simulink model "LMCL"  (R2024b)
settings: Solver=ode4  StartTime=0  StopTime=300  FixedStep=0.01  RelTol=1e-3  AbsTol=1e-6
values from neighbouring files (symbols this model uses):
  C_Alt = pidtune(G_Fz2Alt,'pdf',1)    [controller.m]
  C_phi = pidtune(G_Mx2phi,'pdf',wc)    [controller.m]
  C_psi = pidtune(G_Mz2psi,'pdf',wc)    [controller.m]
  C_tht = pidtune(G_My2tht,'pdf',wc)    [controller.m]
  C_Vx = pidtune(-G_Fx2Vx,'p',0.05)    [controller.m]
  C_Vy = pidtune(-G_Fy2Vy,'p',0.08)    [controller.m]
  C_Vz = pidtune(G_Fz2Vz,'pi',0.05)    [controller.m]
  Ixx = 135582    [initialization.m]
  Iyy = 149140.0    (= 149140)    [initialization.m]
  Izz = 135582    [initialization.m]
  lat_grid = linspace(-90, 90, num_lat)    [initialization.m]
  lon_grid = linspace(-180, 180, num_lon)    [initialization.m]
  moon_dem_table = flipud(raw_data)    [initialization.m]
undefined symbols (not defined in the file or in its folder): datetime, gray, juliandate, Sim3dSensor
libraries: slpidlib x7, sim3dcameralib x3, sim3dlib x2, simulink x2, aerolibtransform2 x2, sharedtransform x1
Description:
  | Apollo Lunar Module Digital Autopilot
settings Model: RequirementInfo=9  SimulationMode=accelerator  PacingRate=1000  Creator=The MathWorks, Inc.  LastModifiedBy=abdma
settings SolverCC: AutoScaleAbsTol=off  AlgebraicLoopSolver=TrustRegion  MaxZcPerStep=1
settings DataIOCC: ExternalInput=op  InitialState=op  SaveFormat=Array  ReturnWorkspaceOutputs=off  SignalLoggingName=logsOut
settings OptimizationCC: BlockReduction=off  ExpressionDepthLimit=2147483647  InitFltsAndDblsToZero=on
settings DebuggingCC: SaveWithParameterizedLinksMsg=none  SignalResolutionControl=TryResolveAllWithWarning  MultiTaskDSMMsg=warning  MultiTaskCondExecSysMsg=none  SigSpecEnsureSampleTimeMsg=none  FcnCallInpInsideContextMsg=warning  UnconnectedInputMsg=warning  UnconnectedOutputMsg=warning  UnconnectedLineMsg=warning  StateNameClashWarn=warning  SFUnexpectedBacktrackingDiag=warning  SFNoUnconditionalDefaultTransitionDiag=warning  SFExecutionAtInitializationDiag=none  ArithmeticOperatorsInVariantConditions=warning
settings HardwareCC: ProdBitPerPointer=32  ProdBitPerSizeT=32  ProdBitPerPtrDiffT=32  ProdLargestAtomicFloat=None  ProdIntDivRoundTo=Undefined  ProdEndianess=Unspecified  ProdWordSize=32  ProdHWDeviceType=Specified
settings ModelReferenceCC: EnableRefExpFcnMdlSchedulingChecks=on  PropagateSignalLabelsOutOfModel=off
settings SFSimCC: SimUseLocalCustomCode=off  SimParseCustomCode=off  CustomCodeUndefinedFunction=UseInterfaceOnly
settings RTWCC: RTWUseLocalCustomCode=off  GPUComputeCapability=3.5  DLArmComputeVersion=19.05
settings CodeAppCC: StateflowObjectComments=on
settings GRTTargetCC: TargetLangStandard=C89/C90 (ANSI)
settings ConfigComp: CovMetricSettings=d  CovSaveCumulativeToWorkspaceVar=on  CovSaveSingleToWorkspaceVar=on  CovExternalEMLEnable=off

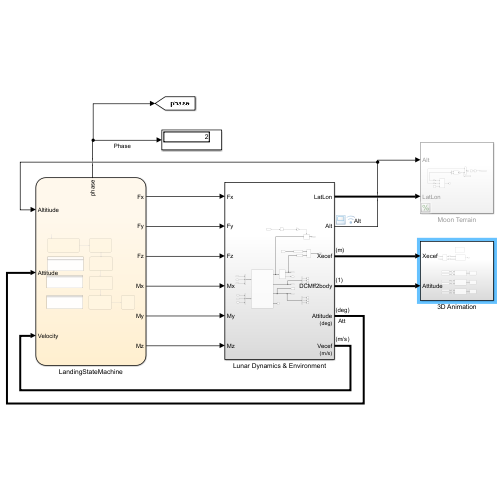
[thumbnail: Simulink's stored preview of the top-level diagram]
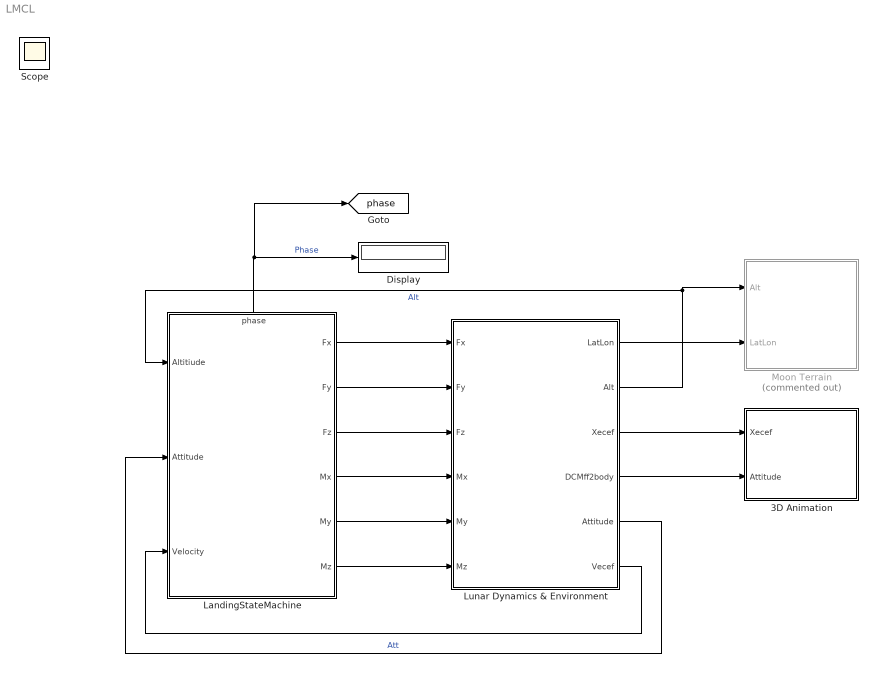
== system LMCL ==
  3D Animation : Subsystem
  Display : Display
  LandingStateMachine : Stateflow chart  TreatAsAtomicUnit=on
      settings: PortSchema="{\"entries\":[{\"content\":{\"sides\":[{\"content\":{\"connectorIds\":[\"In2\",\"In1\",\"In3\"]},\"type\":\"ConnectorPlacement.EquallySpacedRectSide\",\"uuid\":\"b70f077f-5e53-4c11-8b70-291da90a2e92\"},{\"content\":{\"connectorIds\":[\"Out1\",\"Out2\",\"Out3\",\"Out4\",\"Out5\",\"Out6\"],\"side\":\"RIGHT\"},\"type\":\"ConnectorPlacement.EquallySpacedRectSide\",\"uuid\":\"64878038-02c9-47ce-a3b0-eea076ce4bef\"},{\"content\":{\"connectorIds\":[\"Out7\"],\"side\":\"TOP\"},\"type\":\"ConnectorPlacement.EquallySpacedRectSide\",\"uuid\":\"8f914426-e7c7-4385-9703-b406b77ddbb5\"},{\"content\":{\"side\":\"BOTTOM\"},\"type\":\"ConnectorPlacement.EquallySpacedRectSide\",\"uuid\":\"32269b0d-665b-4735-ae33-dac0ab7999d4\"}]},\"type\":\"ConnectorPlacement.EquallySpacedConnector\",\"uuid\":\"201aca57-d29b-4529-a69e-c761b29ced2a\"}],\"packageUris\":[\"http://schema.mathworks.com/mf0/Connector/R2020b\"],\"version\":\"1.0\"}"
  Lunar Dynamics & Environment : Subsystem
  Moon Terrain : Subsystem  Commented=on
  Scope : Scope
  tag scope: phase=global
  wires:
  Lunar Dynamics & Environment/2(Alt) -> LandingStateMachine/2(Altitiude), Moon Terrain/1(Alt)  "Alt"
  Lunar Dynamics & Environment/6(Vecef) -> LandingStateMachine/3(Velocity)
  Lunar Dynamics & Environment/5(Attitude) -> LandingStateMachine/1(Attitude)  "Att"
  LandingStateMachine/1(Fx) -> Lunar Dynamics & Environment/1(Fx)
  LandingStateMachine/2(Fy) -> Lunar Dynamics & Environment/2(Fy)
  LandingStateMachine/3(Fz) -> Lunar Dynamics & Environment/3(Fz)
  LandingStateMachine/4(Mx) -> Lunar Dynamics & Environment/4(Mx)
  LandingStateMachine/5(My) -> Lunar Dynamics & Environment/5(My)
  LandingStateMachine/6(Mz) -> Lunar Dynamics & Environment/6(Mz)
  LandingStateMachine/7(phase) -> [phase], Display/1  "Phase"
  Lunar Dynamics & Environment/1(LatLon) -> Moon Terrain/2(LatLon)
  Lunar Dynamics & Environment/3(Xecef) -> 3D Animation/1(Xecef)
  Lunar Dynamics & Environment/4(DCMff2body) -> 3D Animation/2(Attitude)

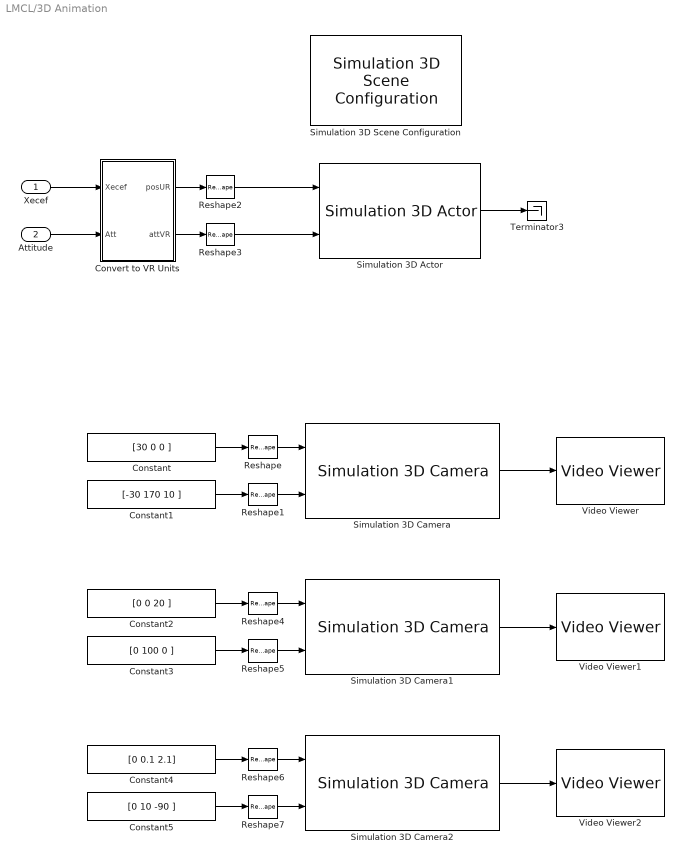
== system LMCL/3D Animation ==
  Xecef : Inport
  Attitude : Inport  Port=2
  Constant : Constant  Value=[30 0 0 ]
  Constant1 : Constant  Value=[-30 170 10 ]
  Constant2 : Constant  Value=[0 0 20 ]
  Constant3 : Constant  Value=[0 100 0 ]
  Constant4 : Constant  Value=[0 0.1 2.1]
  Constant5 : Constant  Value=[0 10 -90 ]
  Convert to VR Units : Subsystem
  Reshape{,1..7} (8 alike) : Reshape  OutputDimensionality=Customize  OutputDimensions=[1,3]
  Simulation 3D Actor : sim3dlib/Simulation 3D Actor  Priority=1  ActorName=LunarModule  ParentName=Scene Origin  Operation=Create at setup  InitScriptText=|  SampleTime=-1  Translation=[10000 10000 10000]  Rotation=[0 0 0]  Scale=[1 1 1]  InputsText=LunarModule.Translation LunarModule.Rotation  aMode=5  ActorTag=LunarModule  ActorType=Sim3dActor  ID=C
      | % Initialize actor
      | Actor.Physics = true;
      | 
      | % Camera that outputs images (optional)
      | camera1 = sim3d.sensors.IdealCamera( ...
      |     'ActorName',"Camera1", ...
      |     "ImageSize",[768, 1024], ...
      |     "HorizontalFieldOfView",60);
      | camera1.Translation = [-3 0 2];
      | add(World, camera1);
      | 
      | % Viewport: this is what changes the view you see
      | createViewport(World, Translation=[-5 0 1], Rotation=[0 0 0]);
  Simulation 3D Camera : sim3dcameralib/Simulation 3D Camera  Priority=1  sensorTag=Sim3dSensor�  sensorId=1  sensorName=Sim3dSensor�  vehTagList={'LunarModule';'Scene Origin'}  vehTag=LunarModule  mountLoc=Origin  offsetFlag=on  tmountOffset=[0, 0, 0]  extTmount=on  rmountOffset=[0, 0, 0]  extRmount=on  FocalLength=[1109, 1109]  OpticalCenter=[640, 360]  ImageSize=[720, 1280]  RadialDistortion=[0, 0]  TangentialDistortion=[0, 0]  SensorSkew=0  DepthOutportEnabled=off  SemanticOutportEnabled=off  TransformOutportEnabled=off  SampleTime=-1  mountPoint=[0 0 0]  mountOrientation=[0 0 0]  aMode=3  ID=1
      settings: LibrarySourceBlock=drivingsim3d/Simulation 3D Camera
  Simulation 3D Camera1 : sim3dcameralib/Simulation 3D Camera  Priority=1  sensorTag=Sim3dSensor�  sensorId=2  sensorName=Sim3dSensor�  vehTagList={'LunarModule';'Scene Origin'}  vehTag=LunarModule  mountLoc=Origin  offsetFlag=on  tmountOffset=[0, 0, 0]  extTmount=on  rmountOffset=[0, 0, 0]  extRmount=on  FocalLength=[1109, 1109]  OpticalCenter=[640, 360]  ImageSize=[720, 1280]  RadialDistortion=[0, 0]  TangentialDistortion=[0, 0]  SensorSkew=0  DepthOutportEnabled=off  SemanticOutportEnabled=off  TransformOutportEnabled=off  SampleTime=-1  mountPoint=[0 0 0]  mountOrientation=[0 0 0]  aMode=3  ID=2
      settings: LibrarySourceBlock=drivingsim3d/Simulation 3D Camera
  Simulation 3D Camera2 : sim3dcameralib/Simulation 3D Camera  Priority=1  sensorTag=Sim3dSensor�  sensorId=3  sensorName=Sim3dSensor�  vehTagList={'LunarModule';'Scene Origin'}  vehTag=LunarModule  mountLoc=Origin  offsetFlag=on  tmountOffset=[0, 0, 0]  extTmount=on  rmountOffset=[0, 0, 0]  extRmount=on  FocalLength=[1109, 1109]  OpticalCenter=[640, 360]  ImageSize=[720, 1280]  RadialDistortion=[0, 0]  TangentialDistortion=[0, 0]  SensorSkew=0  DepthOutportEnabled=off  SemanticOutportEnabled=off  TransformOutportEnabled=off  SampleTime=-1  mountPoint=[0 0 0]  mountOrientation=[0 0 0]  aMode=3  ID=3
      settings: LibrarySourceBlock=drivingsim3d/Simulation 3D Camera
  Simulation 3D Scene Configuration : sim3dlib/Simulation 3D Scene Configuration  Priority=0  ProjectFormat=Unreal Editor  SceneDesc=Empty scene  ProjectName=D:\MATLAB2024b\install\toolbox\shared\sim3d_projects\automotive_project_windows\UE\WindowsNoEditor\VehicleSimulation.exe  ScenePath=/Game/Maps/HwStrght  UEProjPath=C:\Users\abdma\Desktop\Apollo11 Lunar Module Landing\Apollo11\Apollo11.uproject  EnableOpenDRIVE=on  vehTagList={'Custom';'LunarModule';'Scene Origin'}  vehTag=LunarModule  FreeCameraInitialTranslation=[0, 0, 0]  FreeCameraDefaultInitialTranslation=[-6, 0, 2]  FreeCameraInitialRotation=[0, 0, 0]  FreeCameraDefaultInitialRotation=[0, -15, 0]  OpVisEn=off  Ts=0.02  EnableWindow=on  EnableRemoteAccess=off  EnableWeather=off  SunAzimuth=90  SunAltitude=40.0  EnableGeospatialSun=off  Latitude=0  Longitude=0  Date=2023-01-01  Time=10:30:00  GeoTimeZone=-5.0  SunDaylightSaving=off  wind=1  clouds=10  EnableVolumetricClouds=off  CloudCoverage=0  CloudAltitude=6  fog=0  rain=0  RaindropsEffect=off  SnowDensity=0  EnableGeospatial=off  UseTrueOrigin=off  OriginHeight=200  OriginLatitude=40.744652  OriginLongitude=-73.988864  MapStyle=Aerial  AdditionalAssetIDs=[]  UseAdvancedSunSky=off  SolarTime=11  TimeZone=-5  Day=21  Month=9  Year=2022  UseDaylightSavingTime=on  DSTStartDay=10  DSTStartMonth=3  DSTEndDay=3  DSTEndMonth=11  DSTSwitchHour=2  sensorTag=MainCamera1  sensorId=1  sensorName=MainCamera1  mountLoc=Origin  offsetFlag=off  tmountOffset=[0, 0, 0]  rmountOffset=[0, 0, 0]  HorizontalResolution=1280  VerticalResolution=720  HorizontalFOV=60  mountPoint=[0 0 0]  mountOrientation=[0 0 0]  aMode=5  ID=1  GeoTrigger=Inactive
      settings: LibrarySourceBlock=sl3dlib/Simulation 3D/Environment/Simulation 3D Scene Configuration
  Terminator3 : Terminator
  Video Viewer : VideoViewer  colormapValue=gray(256)  FigPos=[769.8 813.2 766.4 300]
  Video Viewer1 : VideoViewer  colormapValue=gray(256)  FigPos=[769.8 405.2 766.4 300]
  Video Viewer2 : VideoViewer  colormapValue=gray(256)  FigPos=[1.8 813.2 766.4 300]
  wires:
  Reshape3/1 -> Simulation 3D Actor/2
  Reshape2/1 -> Simulation 3D Actor/1
  Attitude/1 -> Convert to VR Units/2(Att)
  Xecef/1 -> Convert to VR Units/1(Xecef)
  Simulation 3D Actor/1 -> Terminator3/1
  Convert to VR Units/2(attVR) -> Reshape3/1
  Convert to VR Units/1(posUR) -> Reshape2/1
  Reshape7/1 -> Simulation 3D Camera2/2
  Simulation 3D Camera2/1 -> Video Viewer2/1
  Constant5/1 -> Reshape7/1
  Reshape6/1 -> Simulation 3D Camera2/1
  Reshape1/1 -> Simulation 3D Camera/2
  Reshape/1 -> Simulation 3D Camera/1
  Constant/1 -> Reshape/1
  Constant2/1 -> Reshape4/1
  Reshape4/1 -> Simulation 3D Camera1/1
  Constant4/1 -> Reshape6/1
  Simulation 3D Camera1/1 -> Video Viewer1/1
  Simulation 3D Camera/1 -> Video Viewer/1
  Constant1/1 -> Reshape1/1
  Constant3/1 -> Reshape5/1
  Reshape5/1 -> Simulation 3D Camera1/2

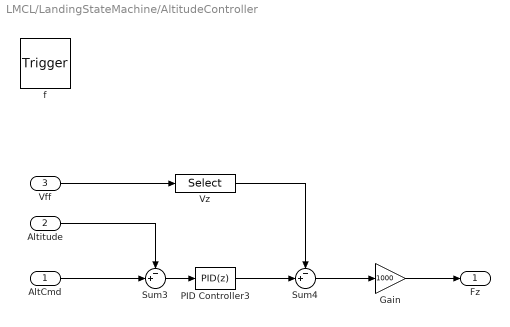
== system LMCL/LandingStateMachine/AltitudeController ==
  AltCmd : Inport  OutDataTypeStr=double  Unit=m  PortDimensions=1
  Altitude : Inport  Port=2  OutDataTypeStr=double  Unit=m  PortDimensions=1
  Vff : Inport  Port=3  OutDataTypeStr=double  Unit=m/s  PortDimensions=[3 1]
  f : TriggerPort  TriggerType=function-call  VariantControl=(inherit)
      settings: CopyFcn=Stateflow.SLINSF.SimulinkMan.removeBlockPreDeleteFcn  PreDeleteFcn=Stateflow.SLINSF.SimulinkMan.unsafePredeleteFcn
  Gain : Gain  Gain=1000
  PID Controller3 : slpidlib/PID Controller  Controller=PID  Form=Parallel  TimeDomain=Discrete-time  UseExternalTs=off  SampleTime=-1  IntegratorMethod=Forward Euler  FilterMethod=Forward Euler  ControllerParametersSource=internal  P=C_Alt.Kp  I=C_Alt.Ki  UseKiTs=off  D=C_Alt.Kd  UseExternalDerivativeSource=off  N=1/C_Alt.Tf  UseFilter=on  TunerSelectOption=Transfer Function Based (PID Tuner App)  InitialConditionSource=internal  InitialConditionForIntegrator=0  InitialConditionForFilter=0  DifferentiatorICPrevScaledInput=0  ExternalReset=none  TrackingMode=off  Kt=1  LimitOutput=on  SatLimitsSource=internal  UpperSaturationLimit=450000  LowerSaturationLimit=-450000  LinearizeAsGain=off  AntiWindupMode=clamping  Kb=1  LimitIntegrator=off  UpperIntegratorSaturationLimit=inf  LowerIntegratorSaturationLimit=-inf  POutMin=[]  POutMax=[]  IOutMin=[]  IOutMax=[]  DOutMin=[]  DOutMax=[]  NOutMin=[]  NOutMax=[]  SumOutMin=[]  SumOutMax=[]  SaturationOutMin=[]  SaturationOutMax=[]  PParamMin=[]  PParamMax=[]  IParamMin=[]  IParamMax=[]  DParamMin=[]  DParamMax=[]  NParamMin=[]  NParamMax=[]  KbParamMin=[]  KbParamMax=[]  KtParamMin=[]  KtParamMax=[]  KbOutMin=[]  KbOutMax=[]  KtOutMin=[]  KtOutMax=[]  IntegratorOutMin=[]  IntegratorOutMax=[]  FilterOutMin=[]  FilterOutMax=[]  SumI1OutMin=[]  SumI1OutMax=[]  SumI2OutMin=[]  SumI2OutMax=[]  SumI3OutMin=[]  SumI3OutMax=[]  SumI4OutMin=[]  SumI4OutMax=[]  SumDOutMin=[]  SumDOutMax=[]  DifferentiatorOutMin=[]  DifferentiatorOutMax=[]  FilterDiffOutCoefMin=[]  FilterDiffOutCoefMax=[]  ReciprocalOutMin=[]  ReciprocalOutMax=[]  SumDenOutMin=[]  SumDenOutMax=[]  SumNumOutMin=[]  SumNumOutMax=[]  DivideOutMin=[]  DivideOutMax=[]  UdiffTsProdOutMin=[]  UdiffTsProdOutMax=[]  NTsProdOutMin=[]  NTsProdOutMax=[]  UintegralTsProdOutMin=[]  UintegralTsProdOutMax=[]  UngainTsProdOutMin=[]  UngainTsProdOutMax=[]  ClampingZeroOutDataTypeStr=Inherit: Inherit via back propagation  ClampingZeroOutMin=[]  ClampingZeroOutMax=[]  FilterDenConstantOutDataTypeStr=Inherit: Inherit via back propagation  FilterDenConstantOutMin=[]  FilterDenConstantOutMax=[]  PCopyOutDataTypeStr=Inherit: Inherit via back propagation  PCopyOutMin=[]  PCopyOutMax=[]  NCopyOutDataTypeStr=Inherit: Inherit via back propagation  NCopyOutMin=[]  NCopyOutMax=[]  IntegratorContinuousStateAttributes=''  IntegratorStateMustResolveToSignalObject=off  IntegratorRTWStateStorageClass=Auto  FilterContinuousStateAttributes=''  FilterStateMustResolveToSignalObject=off  FilterRTWStateStorageClass=Auto  ParallelPVariant=InternalParameters  IdealPVariant=Disabled  IVariant=InternalParameters  DVariant=InternalParameters  IntegratorVariant=Discrete  SatVariant=Enabled  AWVariant=DiscClampingParallel  PCopyVariant=Disabled  TRVariant=Disabled  FdbkBlocksVariant=Forward  IdealPFdbkVariant=Disabled  SatFdbkVariant=Disabled  DerivativeFilterVariant=ForwardEulerFilter  NVariant=InternalParameters  NCopyVariant=Disabled  FilterICVariant=InternalICsFilter  IntegratorICVariant=InternalICs  ExternalResetVariant=Disabled  TRSumVariant=Passthrough  SumFdbkVariant=Disabled  SumVariant=Sum_PID  TsampFilterVariant=InternalTs  TsampNgainVariant=Passthrough  TsampIntegralVariant=Disabled_SignalSpec  ExternalSaturationOutDataTypeStr=Inherit: Same as second input  DerivativeSourceVariant=ErrorSignal  PreIntVariant=InternalPreInt
  Sum3 : Sum  Inputs=-+|
  Sum4 : Sum  Inputs=-+|
  Vz : Selector  InputPortWidth=3  IndexOptions=Index vector (dialog)  Indices=1  OutputSizes=1
  Fz : Outport  OutDataTypeStr=double  Unit=N  PortDimensions=1
  wires:
  Altitude/1 -> Sum3/1
  PID Controller3/1 -> Sum4/2
  Sum3/1 -> PID Controller3/1
  Vff/1 -> Vz/1
  Gain/1 -> Fz/1
  AltCmd/1 -> Sum3/2
  Vz/1 -> Sum4/1
  Sum4/1 -> Gain/1

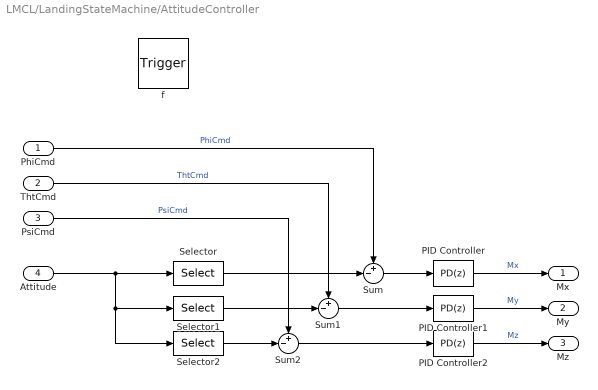
== system LMCL/LandingStateMachine/AttitudeController ==
  PhiCmd : Inport  OutDataTypeStr=double  Unit=deg  PortDimensions=1
  ThtCmd : Inport  Port=2  OutDataTypeStr=double  Unit=deg  PortDimensions=1
  PsiCmd : Inport  Port=3  OutDataTypeStr=double  Unit=deg  PortDimensions=1
  Attitude : Inport  Port=4  OutDataTypeStr=double  Unit=deg  PortDimensions=[3 1]
  f : TriggerPort  TriggerType=function-call  VariantControl=(inherit)
      settings: CopyFcn=Stateflow.SLINSF.SimulinkMan.removeBlockPreDeleteFcn  PreDeleteFcn=Stateflow.SLINSF.SimulinkMan.unsafePredeleteFcn
  PID Controller : slpidlib/PID Controller  Controller=PD  Form=Parallel  TimeDomain=Discrete-time  UseExternalTs=off  SampleTime=-1  IntegratorMethod=Forward Euler  FilterMethod=Forward Euler  ControllerParametersSource=internal  P=C_phi.Kp  I=C_phi.Ki  UseKiTs=off  D=C_phi.Kd  UseExternalDerivativeSource=off  N=1/C_phi.Tf  UseFilter=on  TunerSelectOption=Transfer Function Based (PID Tuner App)  InitialConditionSource=internal  InitialConditionForIntegrator=0  InitialConditionForFilter=0  DifferentiatorICPrevScaledInput=0  ExternalReset=none  TrackingMode=off  Kt=1  LimitOutput=off  SatLimitsSource=internal  UpperSaturationLimit=inf  LowerSaturationLimit=-inf  LinearizeAsGain=on  AntiWindupMode=none  Kb=1  LimitIntegrator=off  UpperIntegratorSaturationLimit=inf  LowerIntegratorSaturationLimit=-inf  POutMin=[]  POutMax=[]  IOutMin=[]  IOutMax=[]  DOutMin=[]  DOutMax=[]  NOutMin=[]  NOutMax=[]  SumOutMin=[]  SumOutMax=[]  SaturationOutMin=[]  SaturationOutMax=[]  PParamMin=[]  PParamMax=[]  IParamMin=[]  IParamMax=[]  DParamMin=[]  DParamMax=[]  NParamMin=[]  NParamMax=[]  KbParamMin=[]  KbParamMax=[]  KtParamMin=[]  KtParamMax=[]  KbOutMin=[]  KbOutMax=[]  KtOutMin=[]  KtOutMax=[]  IntegratorOutMin=[]  IntegratorOutMax=[]  FilterOutMin=[]  FilterOutMax=[]  SumI1OutMin=[]  SumI1OutMax=[]  SumI2OutMin=[]  SumI2OutMax=[]  SumI3OutMin=[]  SumI3OutMax=[]  SumI4OutMin=[]  SumI4OutMax=[]  SumDOutMin=[]  SumDOutMax=[]  DifferentiatorOutMin=[]  DifferentiatorOutMax=[]  FilterDiffOutCoefMin=[]  FilterDiffOutCoefMax=[]  ReciprocalOutMin=[]  ReciprocalOutMax=[]  SumDenOutMin=[]  SumDenOutMax=[]  SumNumOutMin=[]  SumNumOutMax=[]  DivideOutMin=[]  DivideOutMax=[]  UdiffTsProdOutMin=[]  UdiffTsProdOutMax=[]  NTsProdOutMin=[]  NTsProdOutMax=[]  UintegralTsProdOutMin=[]  UintegralTsProdOutMax=[]  UngainTsProdOutMin=[]  UngainTsProdOutMax=[]  ClampingZeroOutDataTypeStr=Inherit: Inherit via back propagation  ClampingZeroOutMin=[]  ClampingZeroOutMax=[]  FilterDenConstantOutDataTypeStr=Inherit: Inherit via back propagation  FilterDenConstantOutMin=[]  FilterDenConstantOutMax=[]  PCopyOutDataTypeStr=Inherit: Inherit via back propagation  PCopyOutMin=[]  PCopyOutMax=[]  NCopyOutDataTypeStr=Inherit: Inherit via back propagation  NCopyOutMin=[]  NCopyOutMax=[]  IntegratorContinuousStateAttributes=''  IntegratorStateMustResolveToSignalObject=off  IntegratorRTWStateStorageClass=Auto  FilterContinuousStateAttributes=''  FilterStateMustResolveToSignalObject=off  FilterRTWStateStorageClass=Auto  ParallelPVariant=InternalParameters  IdealPVariant=Disabled  IVariant=Disabled  DVariant=InternalParameters  IntegratorVariant=Disabled  SatVariant=Disabled  AWVariant=Disabled  PCopyVariant=Disabled  TRVariant=Disabled  FdbkBlocksVariant=Forward  IdealPFdbkVariant=Disabled  SatFdbkVariant=Disabled  DerivativeFilterVariant=ForwardEulerFilter  NVariant=InternalParameters  NCopyVariant=Disabled  FilterICVariant=InternalICsFilter  IntegratorICVariant=Disabled  ExternalResetVariant=Disabled  TRSumVariant=Passthrough  SumFdbkVariant=Disabled  SumVariant=Sum_PD  TsampFilterVariant=InternalTs  TsampNgainVariant=Passthrough  TsampIntegralVariant=Disabled_SignalSpec  ExternalSaturationOutDataTypeStr=Inherit: Same as second input  DerivativeSourceVariant=ErrorSignal  PreIntVariant=InternalPreInt
  PID Controller1 : slpidlib/PID Controller  Controller=PD  Form=Parallel  TimeDomain=Discrete-time  UseExternalTs=off  SampleTime=-1  IntegratorMethod=Forward Euler  FilterMethod=Forward Euler  ControllerParametersSource=internal  P=C_tht.Kp  I=C_tht.Ki  UseKiTs=off  D=C_tht.Kd  UseExternalDerivativeSource=off  N=1/C_tht.Tf  UseFilter=on  TunerSelectOption=Transfer Function Based (PID Tuner App)  InitialConditionSource=internal  InitialConditionForIntegrator=0  InitialConditionForFilter=0  DifferentiatorICPrevScaledInput=0  ExternalReset=none  TrackingMode=off  Kt=1  LimitOutput=off  SatLimitsSource=internal  UpperSaturationLimit=inf  LowerSaturationLimit=-inf  LinearizeAsGain=on  AntiWindupMode=none  Kb=1  LimitIntegrator=off  UpperIntegratorSaturationLimit=inf  LowerIntegratorSaturationLimit=-inf  POutMin=[]  POutMax=[]  IOutMin=[]  IOutMax=[]  DOutMin=[]  DOutMax=[]  NOutMin=[]  NOutMax=[]  SumOutMin=[]  SumOutMax=[]  SaturationOutMin=[]  SaturationOutMax=[]  PParamMin=[]  PParamMax=[]  IParamMin=[]  IParamMax=[]  DParamMin=[]  DParamMax=[]  NParamMin=[]  NParamMax=[]  KbParamMin=[]  KbParamMax=[]  KtParamMin=[]  KtParamMax=[]  KbOutMin=[]  KbOutMax=[]  KtOutMin=[]  KtOutMax=[]  IntegratorOutMin=[]  IntegratorOutMax=[]  FilterOutMin=[]  FilterOutMax=[]  SumI1OutMin=[]  SumI1OutMax=[]  SumI2OutMin=[]  SumI2OutMax=[]  SumI3OutMin=[]  SumI3OutMax=[]  SumI4OutMin=[]  SumI4OutMax=[]  SumDOutMin=[]  SumDOutMax=[]  DifferentiatorOutMin=[]  DifferentiatorOutMax=[]  FilterDiffOutCoefMin=[]  FilterDiffOutCoefMax=[]  ReciprocalOutMin=[]  ReciprocalOutMax=[]  SumDenOutMin=[]  SumDenOutMax=[]  SumNumOutMin=[]  SumNumOutMax=[]  DivideOutMin=[]  DivideOutMax=[]  UdiffTsProdOutMin=[]  UdiffTsProdOutMax=[]  NTsProdOutMin=[]  NTsProdOutMax=[]  UintegralTsProdOutMin=[]  UintegralTsProdOutMax=[]  UngainTsProdOutMin=[]  UngainTsProdOutMax=[]  ClampingZeroOutDataTypeStr=Inherit: Inherit via back propagation  ClampingZeroOutMin=[]  ClampingZeroOutMax=[]  FilterDenConstantOutDataTypeStr=Inherit: Inherit via back propagation  FilterDenConstantOutMin=[]  FilterDenConstantOutMax=[]  PCopyOutDataTypeStr=Inherit: Inherit via back propagation  PCopyOutMin=[]  PCopyOutMax=[]  NCopyOutDataTypeStr=Inherit: Inherit via back propagation  NCopyOutMin=[]  NCopyOutMax=[]  IntegratorContinuousStateAttributes=''  IntegratorStateMustResolveToSignalObject=off  IntegratorRTWStateStorageClass=Auto  FilterContinuousStateAttributes=''  FilterStateMustResolveToSignalObject=off  FilterRTWStateStorageClass=Auto  ParallelPVariant=InternalParameters  IdealPVariant=Disabled  IVariant=Disabled  DVariant=InternalParameters  IntegratorVariant=Disabled  SatVariant=Disabled  AWVariant=Disabled  PCopyVariant=Disabled  TRVariant=Disabled  FdbkBlocksVariant=Forward  IdealPFdbkVariant=Disabled  SatFdbkVariant=Disabled  DerivativeFilterVariant=ForwardEulerFilter  NVariant=InternalParameters  NCopyVariant=Disabled  FilterICVariant=InternalICsFilter  IntegratorICVariant=Disabled  ExternalResetVariant=Disabled  TRSumVariant=Passthrough  SumFdbkVariant=Disabled  SumVariant=Sum_PD  TsampFilterVariant=InternalTs  TsampNgainVariant=Passthrough  TsampIntegralVariant=Disabled_SignalSpec  ExternalSaturationOutDataTypeStr=Inherit: Same as second input  DerivativeSourceVariant=ErrorSignal  PreIntVariant=InternalPreInt
  PID Controller2 : slpidlib/PID Controller  Controller=PD  Form=Parallel  TimeDomain=Discrete-time  UseExternalTs=off  SampleTime=-1  IntegratorMethod=Forward Euler  FilterMethod=Forward Euler  ControllerParametersSource=internal  P=C_psi.Kp  I=C_psi.Ki  UseKiTs=off  D=C_psi.Kd  UseExternalDerivativeSource=off  N=1/C_psi.Tf  UseFilter=on  TunerSelectOption=Transfer Function Based (PID Tuner App)  InitialConditionSource=internal  InitialConditionForIntegrator=0  InitialConditionForFilter=0  DifferentiatorICPrevScaledInput=0  ExternalReset=none  TrackingMode=off  Kt=1  LimitOutput=off  SatLimitsSource=internal  UpperSaturationLimit=inf  LowerSaturationLimit=-inf  LinearizeAsGain=on  AntiWindupMode=none  Kb=1  LimitIntegrator=off  UpperIntegratorSaturationLimit=inf  LowerIntegratorSaturationLimit=-inf  POutMin=[]  POutMax=[]  IOutMin=[]  IOutMax=[]  DOutMin=[]  DOutMax=[]  NOutMin=[]  NOutMax=[]  SumOutMin=[]  SumOutMax=[]  SaturationOutMin=[]  SaturationOutMax=[]  PParamMin=[]  PParamMax=[]  IParamMin=[]  IParamMax=[]  DParamMin=[]  DParamMax=[]  NParamMin=[]  NParamMax=[]  KbParamMin=[]  KbParamMax=[]  KtParamMin=[]  KtParamMax=[]  KbOutMin=[]  KbOutMax=[]  KtOutMin=[]  KtOutMax=[]  IntegratorOutMin=[]  IntegratorOutMax=[]  FilterOutMin=[]  FilterOutMax=[]  SumI1OutMin=[]  SumI1OutMax=[]  SumI2OutMin=[]  SumI2OutMax=[]  SumI3OutMin=[]  SumI3OutMax=[]  SumI4OutMin=[]  SumI4OutMax=[]  SumDOutMin=[]  SumDOutMax=[]  DifferentiatorOutMin=[]  DifferentiatorOutMax=[]  FilterDiffOutCoefMin=[]  FilterDiffOutCoefMax=[]  ReciprocalOutMin=[]  ReciprocalOutMax=[]  SumDenOutMin=[]  SumDenOutMax=[]  SumNumOutMin=[]  SumNumOutMax=[]  DivideOutMin=[]  DivideOutMax=[]  UdiffTsProdOutMin=[]  UdiffTsProdOutMax=[]  NTsProdOutMin=[]  NTsProdOutMax=[]  UintegralTsProdOutMin=[]  UintegralTsProdOutMax=[]  UngainTsProdOutMin=[]  UngainTsProdOutMax=[]  ClampingZeroOutDataTypeStr=Inherit: Inherit via back propagation  ClampingZeroOutMin=[]  ClampingZeroOutMax=[]  FilterDenConstantOutDataTypeStr=Inherit: Inherit via back propagation  FilterDenConstantOutMin=[]  FilterDenConstantOutMax=[]  PCopyOutDataTypeStr=Inherit: Inherit via back propagation  PCopyOutMin=[]  PCopyOutMax=[]  NCopyOutDataTypeStr=Inherit: Inherit via back propagation  NCopyOutMin=[]  NCopyOutMax=[]  IntegratorContinuousStateAttributes=''  IntegratorStateMustResolveToSignalObject=off  IntegratorRTWStateStorageClass=Auto  FilterContinuousStateAttributes=''  FilterStateMustResolveToSignalObject=off  FilterRTWStateStorageClass=Auto  ParallelPVariant=InternalParameters  IdealPVariant=Disabled  IVariant=Disabled  DVariant=InternalParameters  IntegratorVariant=Disabled  SatVariant=Disabled  AWVariant=Disabled  PCopyVariant=Disabled  TRVariant=Disabled  FdbkBlocksVariant=Forward  IdealPFdbkVariant=Disabled  SatFdbkVariant=Disabled  DerivativeFilterVariant=ForwardEulerFilter  NVariant=InternalParameters  NCopyVariant=Disabled  FilterICVariant=InternalICsFilter  IntegratorICVariant=Disabled  ExternalResetVariant=Disabled  TRSumVariant=Passthrough  SumFdbkVariant=Disabled  SumVariant=Sum_PD  TsampFilterVariant=InternalTs  TsampNgainVariant=Passthrough  TsampIntegralVariant=Disabled_SignalSpec  ExternalSaturationOutDataTypeStr=Inherit: Same as second input  DerivativeSourceVariant=ErrorSignal  PreIntVariant=InternalPreInt
  Selector : Selector  InputPortWidth=3  IndexOptions=Index vector (dialog)  Indices=1  OutputSizes=1
  Selector1 : Selector  InputPortWidth=3  IndexOptions=Index vector (dialog)  Indices=2  OutputSizes=1
  Selector2 : Selector  InputPortWidth=3  IndexOptions=Index vector (dialog)  Indices=3  OutputSizes=1
  Sum : Sum  Inputs=+-|
  Sum1 : Sum  Inputs=+-|
  Sum2 : Sum  Inputs=+-|
  Mx : Outport  OutDataTypeStr=double  Unit=N*m  PortDimensions=1
  My : Outport  Port=2  OutDataTypeStr=double  Unit=N*m  PortDimensions=1
  Mz : Outport  Port=3  OutDataTypeStr=double  Unit=N*m
  wires:
  PhiCmd/1 -> Sum/1  "PhiCmd"
  Selector2/1 -> Sum2/2
  Sum2/1 -> PID Controller2/1
  Sum1/1 -> PID Controller1/1
  Sum/1 -> PID Controller/1
  ThtCmd/1 -> Sum1/1  "ThtCmd"
  Selector1/1 -> Sum1/2
  Attitude/1 -> Selector2/1, Selector1/1, Selector/1
  PsiCmd/1 -> Sum2/1  "PsiCmd"
  Selector/1 -> Sum/2
  PID Controller1/1 -> My/1  "My"
  PID Controller/1 -> Mx/1  "Mx"
  PID Controller2/1 -> Mz/1  "Mz"

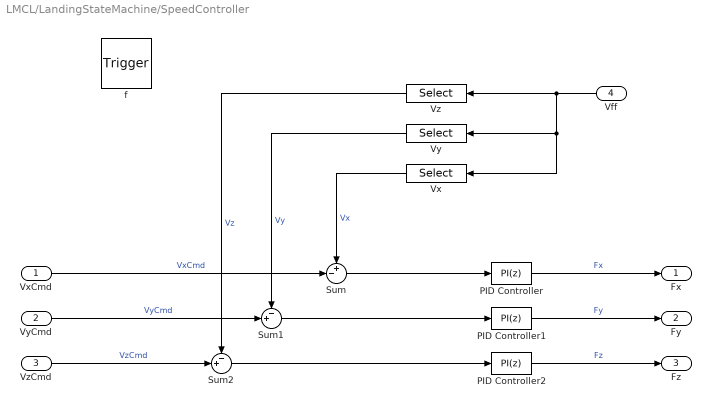
== system LMCL/LandingStateMachine/SpeedController ==
  VxCmd : Inport  OutDataTypeStr=double  Unit=m/s  PortDimensions=1
  VyCmd : Inport  Port=2  OutDataTypeStr=double  Unit=m/s  PortDimensions=1
  VzCmd : Inport  Port=3  OutDataTypeStr=double  Unit=m/s  PortDimensions=1
  Vff : Inport  Port=4  OutDataTypeStr=double  Unit=m/s  PortDimensions=[3 1]
  f : TriggerPort  TriggerType=function-call  VariantControl=(inherit)
      settings: CopyFcn=Stateflow.SLINSF.SimulinkMan.removeBlockPreDeleteFcn  PreDeleteFcn=Stateflow.SLINSF.SimulinkMan.unsafePredeleteFcn
  PID Controller : slpidlib/PID Controller  Controller=PI  Form=Parallel  TimeDomain=Discrete-time  UseExternalTs=off  SampleTime=-1  IntegratorMethod=Forward Euler  FilterMethod=Forward Euler  ControllerParametersSource=internal  P=C_Vx.Kp  I=C_Vx.Ki  UseKiTs=off  D=0  UseExternalDerivativeSource=off  N=100  UseFilter=on  TunerSelectOption=Transfer Function Based (PID Tuner App)  InitialConditionSource=internal  InitialConditionForIntegrator=0  InitialConditionForFilter=0  DifferentiatorICPrevScaledInput=0  ExternalReset=none  TrackingMode=off  Kt=1  LimitOutput=on  SatLimitsSource=internal  UpperSaturationLimit=450000  LowerSaturationLimit=-450000  LinearizeAsGain=off  AntiWindupMode=clamping  Kb=1  LimitIntegrator=off  UpperIntegratorSaturationLimit=inf  LowerIntegratorSaturationLimit=-inf  POutMin=[]  POutMax=[]  IOutMin=[]  IOutMax=[]  DOutMin=[]  DOutMax=[]  NOutMin=[]  NOutMax=[]  SumOutMin=[]  SumOutMax=[]  SaturationOutMin=[]  SaturationOutMax=[]  PParamMin=[]  PParamMax=[]  IParamMin=[]  IParamMax=[]  DParamMin=[]  DParamMax=[]  NParamMin=[]  NParamMax=[]  KbParamMin=[]  KbParamMax=[]  KtParamMin=[]  KtParamMax=[]  KbOutMin=[]  KbOutMax=[]  KtOutMin=[]  KtOutMax=[]  IntegratorOutMin=[]  IntegratorOutMax=[]  FilterOutMin=[]  FilterOutMax=[]  SumI1OutMin=[]  SumI1OutMax=[]  SumI2OutMin=[]  SumI2OutMax=[]  SumI3OutMin=[]  SumI3OutMax=[]  SumI4OutMin=[]  SumI4OutMax=[]  SumDOutMin=[]  SumDOutMax=[]  DifferentiatorOutMin=[]  DifferentiatorOutMax=[]  FilterDiffOutCoefMin=[]  FilterDiffOutCoefMax=[]  ReciprocalOutMin=[]  ReciprocalOutMax=[]  SumDenOutMin=[]  SumDenOutMax=[]  SumNumOutMin=[]  SumNumOutMax=[]  DivideOutMin=[]  DivideOutMax=[]  UdiffTsProdOutMin=[]  UdiffTsProdOutMax=[]  NTsProdOutMin=[]  NTsProdOutMax=[]  UintegralTsProdOutMin=[]  UintegralTsProdOutMax=[]  UngainTsProdOutMin=[]  UngainTsProdOutMax=[]  ClampingZeroOutDataTypeStr=Inherit: Inherit via back propagation  ClampingZeroOutMin=[]  ClampingZeroOutMax=[]  FilterDenConstantOutDataTypeStr=Inherit: Inherit via back propagation  FilterDenConstantOutMin=[]  FilterDenConstantOutMax=[]  PCopyOutDataTypeStr=Inherit: Inherit via back propagation  PCopyOutMin=[]  PCopyOutMax=[]  NCopyOutDataTypeStr=Inherit: Inherit via back propagation  NCopyOutMin=[]  NCopyOutMax=[]  IntegratorContinuousStateAttributes=''  IntegratorStateMustResolveToSignalObject=off  IntegratorRTWStateStorageClass=Auto  FilterContinuousStateAttributes=''  FilterStateMustResolveToSignalObject=off  FilterRTWStateStorageClass=Auto  ParallelPVariant=InternalParameters  IdealPVariant=Disabled  IVariant=InternalParameters  DVariant=Disabled  IntegratorVariant=Discrete  SatVariant=Enabled  AWVariant=DiscClampingParallel  PCopyVariant=Disabled  TRVariant=Disabled  FdbkBlocksVariant=Forward  IdealPFdbkVariant=Disabled  SatFdbkVariant=Disabled  DerivativeFilterVariant=Disabled  NVariant=Disabled  NCopyVariant=Disabled_SignalSpec  FilterICVariant=Disabled  IntegratorICVariant=InternalICs  ExternalResetVariant=Disabled  TRSumVariant=Passthrough  SumFdbkVariant=Disabled  SumVariant=Sum_PI  TsampFilterVariant=InternalTs  TsampNgainVariant=Passthrough  TsampIntegralVariant=Disabled_SignalSpec  ExternalSaturationOutDataTypeStr=Inherit: Same as second input  DerivativeSourceVariant=Disabled  PreIntVariant=InternalPreInt
  PID Controller1 : slpidlib/PID Controller  Controller=PI  Form=Parallel  TimeDomain=Discrete-time  UseExternalTs=off  SampleTime=-1  IntegratorMethod=Forward Euler  FilterMethod=Forward Euler  ControllerParametersSource=internal  P=C_Vy.Kp  I=C_Vy.Ki  UseKiTs=off  D=0  UseExternalDerivativeSource=off  N=100  UseFilter=on  TunerSelectOption=Transfer Function Based (PID Tuner App)  InitialConditionSource=internal  InitialConditionForIntegrator=0  InitialConditionForFilter=0  DifferentiatorICPrevScaledInput=0  ExternalReset=none  TrackingMode=off  Kt=1  LimitOutput=on  SatLimitsSource=internal  UpperSaturationLimit=450000  LowerSaturationLimit=-450000  LinearizeAsGain=off  AntiWindupMode=clamping  Kb=1  LimitIntegrator=off  UpperIntegratorSaturationLimit=inf  LowerIntegratorSaturationLimit=-inf  POutMin=[]  POutMax=[]  IOutMin=[]  IOutMax=[]  DOutMin=[]  DOutMax=[]  NOutMin=[]  NOutMax=[]  SumOutMin=[]  SumOutMax=[]  SaturationOutMin=[]  SaturationOutMax=[]  PParamMin=[]  PParamMax=[]  IParamMin=[]  IParamMax=[]  DParamMin=[]  DParamMax=[]  NParamMin=[]  NParamMax=[]  KbParamMin=[]  KbParamMax=[]  KtParamMin=[]  KtParamMax=[]  KbOutMin=[]  KbOutMax=[]  KtOutMin=[]  KtOutMax=[]  IntegratorOutMin=[]  IntegratorOutMax=[]  FilterOutMin=[]  FilterOutMax=[]  SumI1OutMin=[]  SumI1OutMax=[]  SumI2OutMin=[]  SumI2OutMax=[]  SumI3OutMin=[]  SumI3OutMax=[]  SumI4OutMin=[]  SumI4OutMax=[]  SumDOutMin=[]  SumDOutMax=[]  DifferentiatorOutMin=[]  DifferentiatorOutMax=[]  FilterDiffOutCoefMin=[]  FilterDiffOutCoefMax=[]  ReciprocalOutMin=[]  ReciprocalOutMax=[]  SumDenOutMin=[]  SumDenOutMax=[]  SumNumOutMin=[]  SumNumOutMax=[]  DivideOutMin=[]  DivideOutMax=[]  UdiffTsProdOutMin=[]  UdiffTsProdOutMax=[]  NTsProdOutMin=[]  NTsProdOutMax=[]  UintegralTsProdOutMin=[]  UintegralTsProdOutMax=[]  UngainTsProdOutMin=[]  UngainTsProdOutMax=[]  ClampingZeroOutDataTypeStr=Inherit: Inherit via back propagation  ClampingZeroOutMin=[]  ClampingZeroOutMax=[]  FilterDenConstantOutDataTypeStr=Inherit: Inherit via back propagation  FilterDenConstantOutMin=[]  FilterDenConstantOutMax=[]  PCopyOutDataTypeStr=Inherit: Inherit via back propagation  PCopyOutMin=[]  PCopyOutMax=[]  NCopyOutDataTypeStr=Inherit: Inherit via back propagation  NCopyOutMin=[]  NCopyOutMax=[]  IntegratorContinuousStateAttributes=''  IntegratorStateMustResolveToSignalObject=off  IntegratorRTWStateStorageClass=Auto  FilterContinuousStateAttributes=''  FilterStateMustResolveToSignalObject=off  FilterRTWStateStorageClass=Auto  ParallelPVariant=InternalParameters  IdealPVariant=Disabled  IVariant=InternalParameters  DVariant=Disabled  IntegratorVariant=Discrete  SatVariant=Enabled  AWVariant=DiscClampingParallel  PCopyVariant=Disabled  TRVariant=Disabled  FdbkBlocksVariant=Forward  IdealPFdbkVariant=Disabled  SatFdbkVariant=Disabled  DerivativeFilterVariant=Disabled  NVariant=Disabled  NCopyVariant=Disabled_SignalSpec  FilterICVariant=Disabled  IntegratorICVariant=InternalICs  ExternalResetVariant=Disabled  TRSumVariant=Passthrough  SumFdbkVariant=Disabled  SumVariant=Sum_PI  TsampFilterVariant=InternalTs  TsampNgainVariant=Passthrough  TsampIntegralVariant=Disabled_SignalSpec  ExternalSaturationOutDataTypeStr=Inherit: Same as second input  DerivativeSourceVariant=Disabled  PreIntVariant=InternalPreInt
  PID Controller2 : slpidlib/PID Controller  Controller=PI  Form=Parallel  TimeDomain=Discrete-time  UseExternalTs=off  SampleTime=-1  IntegratorMethod=Forward Euler  FilterMethod=Forward Euler  ControllerParametersSource=internal  P=C_Vz.Kp  I=C_Vz.Ki  UseKiTs=off  D=0  UseExternalDerivativeSource=off  N=100  UseFilter=on  TunerSelectOption=Transfer Function Based (PID Tuner App)  InitialConditionSource=internal  InitialConditionForIntegrator=0  InitialConditionForFilter=0  DifferentiatorICPrevScaledInput=0  ExternalReset=none  TrackingMode=off  Kt=1  LimitOutput=on  SatLimitsSource=internal  UpperSaturationLimit=450000  LowerSaturationLimit=-450000  LinearizeAsGain=off  AntiWindupMode=clamping  Kb=1  LimitIntegrator=off  UpperIntegratorSaturationLimit=inf  LowerIntegratorSaturationLimit=-inf  POutMin=[]  POutMax=[]  IOutMin=[]  IOutMax=[]  DOutMin=[]  DOutMax=[]  NOutMin=[]  NOutMax=[]  SumOutMin=[]  SumOutMax=[]  SaturationOutMin=[]  SaturationOutMax=[]  PParamMin=[]  PParamMax=[]  IParamMin=[]  IParamMax=[]  DParamMin=[]  DParamMax=[]  NParamMin=[]  NParamMax=[]  KbParamMin=[]  KbParamMax=[]  KtParamMin=[]  KtParamMax=[]  KbOutMin=[]  KbOutMax=[]  KtOutMin=[]  KtOutMax=[]  IntegratorOutMin=[]  IntegratorOutMax=[]  FilterOutMin=[]  FilterOutMax=[]  SumI1OutMin=[]  SumI1OutMax=[]  SumI2OutMin=[]  SumI2OutMax=[]  SumI3OutMin=[]  SumI3OutMax=[]  SumI4OutMin=[]  SumI4OutMax=[]  SumDOutMin=[]  SumDOutMax=[]  DifferentiatorOutMin=[]  DifferentiatorOutMax=[]  FilterDiffOutCoefMin=[]  FilterDiffOutCoefMax=[]  ReciprocalOutMin=[]  ReciprocalOutMax=[]  SumDenOutMin=[]  SumDenOutMax=[]  SumNumOutMin=[]  SumNumOutMax=[]  DivideOutMin=[]  DivideOutMax=[]  UdiffTsProdOutMin=[]  UdiffTsProdOutMax=[]  NTsProdOutMin=[]  NTsProdOutMax=[]  UintegralTsProdOutMin=[]  UintegralTsProdOutMax=[]  UngainTsProdOutMin=[]  UngainTsProdOutMax=[]  ClampingZeroOutDataTypeStr=Inherit: Inherit via back propagation  ClampingZeroOutMin=[]  ClampingZeroOutMax=[]  FilterDenConstantOutDataTypeStr=Inherit: Inherit via back propagation  FilterDenConstantOutMin=[]  FilterDenConstantOutMax=[]  PCopyOutDataTypeStr=Inherit: Inherit via back propagation  PCopyOutMin=[]  PCopyOutMax=[]  NCopyOutDataTypeStr=Inherit: Inherit via back propagation  NCopyOutMin=[]  NCopyOutMax=[]  IntegratorContinuousStateAttributes=''  IntegratorStateMustResolveToSignalObject=off  IntegratorRTWStateStorageClass=Auto  FilterContinuousStateAttributes=''  FilterStateMustResolveToSignalObject=off  FilterRTWStateStorageClass=Auto  ParallelPVariant=InternalParameters  IdealPVariant=Disabled  IVariant=InternalParameters  DVariant=Disabled  IntegratorVariant=Discrete  SatVariant=Enabled  AWVariant=DiscClampingParallel  PCopyVariant=Disabled  TRVariant=Disabled  FdbkBlocksVariant=Forward  IdealPFdbkVariant=Disabled  SatFdbkVariant=Disabled  DerivativeFilterVariant=Disabled  NVariant=Disabled  NCopyVariant=Disabled_SignalSpec  FilterICVariant=Disabled  IntegratorICVariant=InternalICs  ExternalResetVariant=Disabled  TRSumVariant=Passthrough  SumFdbkVariant=Disabled  SumVariant=Sum_PI  TsampFilterVariant=InternalTs  TsampNgainVariant=Passthrough  TsampIntegralVariant=Disabled_SignalSpec  ExternalSaturationOutDataTypeStr=Inherit: Same as second input  DerivativeSourceVariant=Disabled  PreIntVariant=InternalPreInt
  Sum : Sum  Inputs=+-|
  Sum1 : Sum  Inputs=-+|
  Sum2 : Sum  Inputs=-+|
  Vx : Selector  InputPortWidth=3  IndexOptions=Index vector (dialog)  Indices=3  OutputSizes=1
  Vy : Selector  InputPortWidth=3  IndexOptions=Index vector (dialog)  Indices=2  OutputSizes=1
  Vz : Selector  InputPortWidth=3  IndexOptions=Index vector (dialog)  Indices=1  OutputSizes=1
  Fx : Outport  OutDataTypeStr=double  Unit=N  PortDimensions=1
  Fy : Outport  Port=2  OutDataTypeStr=double  Unit=N  PortDimensions=1
  Fz : Outport  Port=3  OutDataTypeStr=double  Unit=N  PortDimensions=1
  wires:
  Vx/1 -> Sum/1  "Vx"
  VyCmd/1 -> Sum1/2  "VyCmd"
  PID Controller2/1 -> Fz/1  "Fz"
  Sum2/1 -> PID Controller2/1
  PID Controller/1 -> Fx/1  "Fx"
  PID Controller1/1 -> Fy/1  "Fy"
  Vff/1 -> Vz/1, Vx/1, Vy/1
  VxCmd/1 -> Sum/2  "VxCmd"
  Sum/1 -> PID Controller/1
  VzCmd/1 -> Sum2/2  "VzCmd"
  Vz/1 -> Sum2/1  "Vz"
  Vy/1 -> Sum1/1  "Vy"
  Sum1/1 -> PID Controller1/1

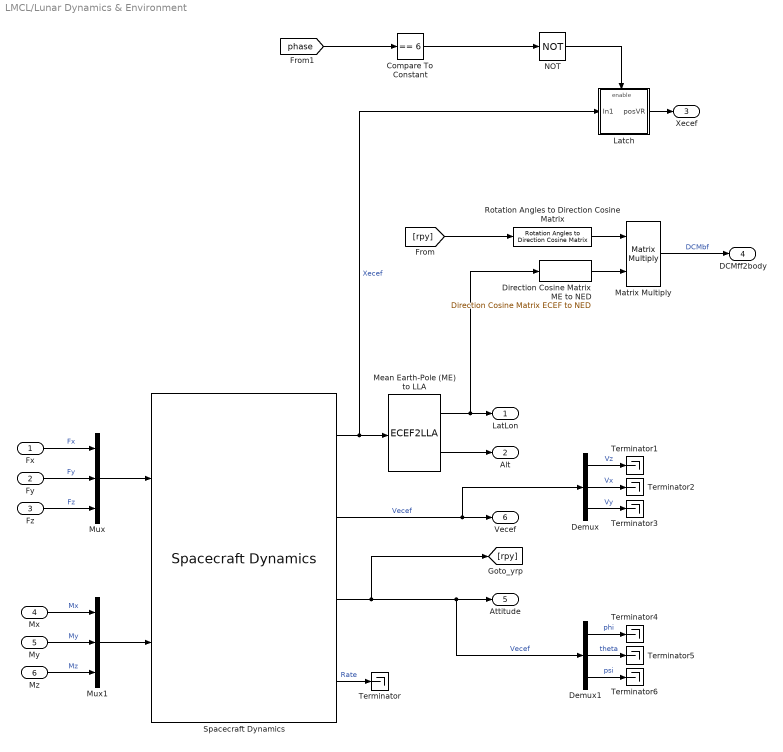
== system LMCL/Lunar Dynamics & Environment ==
  Fx : Inport
  Fy : Inport  Port=2
  Fz : Inport  Port=3
  Mx : Inport  Port=4
  My : Inport  Port=5
  Mz : Inport  Port=6
  Compare To Constant : simulink/Logic and Bit Operations/Compare To Constant  relop===  const=6  OutDataTypeStr=boolean
  Demux : Demux  Outputs=3
  Demux1 : Demux  Outputs=3
  Direction Cosine Matrix ME to NED : aerolibtransform2/Direction Cosine Matrix ECEF to NED
  Latch : Subsystem  TreatAsAtomicUnit=on
  Matrix Multiply : Product  Multiplication=Matrix(*)
  Mean Earth-Pole (ME) to LLA : ECEF2LLA  ptype=Custom  F=0.0012  R=17.374e5
  Mux : Mux  Inputs=3
  Mux1 : Mux  Inputs=3
  NOT : Logic  Operator=NOT  IconShape=distinctive  AllPortsSameDT=off  OutDataTypeStr=boolean
  Rotation Angles to Direction Cosine Matrix : sharedtransform/Rotation Angles to Direction Cosine Matrix  rotationOrder=ZXY  aMode=aMode
  Spacecraft Dynamics : SpacecraftDynamics  accelFrame=Fixed-frame  outportFrame=Fixed-frame  startDate=juliandate(datetime('20-Jul-1969 19:08:44'))  dateOut=off  mass=mass  inertia=diag([Ixx,Iyy,Izz])  stateFormatNum=Fixed-frame state vector  inertialPosition=Xicrf0  inertialVelocity=Vicrf0  fixedPosition=Xff0  fixedVelocity=Vff0  attitudeFrame=NED  attitudeFormat=Euler angles  attitude=Att0  rotationOrder=XYZ  attitudeRate=Omg0  useGravGrad=off  centralBody=Moon  shDegree=60
      settings: AttributesFormatString=|
      | Central Body: %<centralBody>
      | Gravity Model: %<gravityModel> (%<moonSH>)
  Terminator{,1..6} (7 alike) : Terminator
  LatLon : Outport  VectorParamsAs1DForOutWhenUnconnected=off
  Alt : Outport  Port=2  VectorParamsAs1DForOutWhenUnconnected=off
  Xecef : Outport  Port=3
  DCMff2body : Outport  Port=4
  Attitude : Outport  Port=5  Unit=deg  VectorParamsAs1DForOutWhenUnconnected=off
  Vecef : Outport  Port=6  Unit=m/s
  wires:
  Mean Earth-Pole (ME) to LLA/2 -> Alt/1
  Spacecraft Dynamics/1 -> Latch/1(In1), Mean Earth-Pole (ME) to LLA/1  "Xecef"
  Mx/1 -> Mux1/1  "Mx"
  Mux1/1 -> Spacecraft Dynamics/2
  Mux/1 -> Spacecraft Dynamics/1
  Fx/1 -> Mux/1  "Fx"
  Fz/1 -> Mux/3  "Fz"
  My/1 -> Mux1/2  "My"
  Mz/1 -> Mux1/3  "Mz"
  Fy/1 -> Mux/2  "Fy"
  Matrix Multiply/1 -> DCMff2body/1  "DCMbf"
  Rotation Angles to Direction Cosine Matrix/1 -> Matrix Multiply/1
  [rpy] -> Rotation Angles to Direction Cosine Matrix/1
  Mean Earth-Pole (ME) to LLA/1 -> Direction Cosine Matrix ME to NED/1, LatLon/1
  Direction Cosine Matrix ME to NED/1 -> Matrix Multiply/2
  Spacecraft Dynamics/2 -> Demux/1, Vecef/1  "Vecef"
  Spacecraft Dynamics/4 -> Terminator/1  "Rate"
  Demux/1 -> Terminator1/1  "Vz"
  Demux/2 -> Terminator2/1  "Vx"
  Demux/3 -> Terminator3/1  "Vy"
  Compare To Constant/1 -> NOT/1
  [phase] -> Compare To Constant/1
  NOT/1 -> Latch/Enable
  Latch/1(posVR) -> Xecef/1
  Demux1/3 -> Terminator6/1  "psi"
  Demux1/2 -> Terminator5/1  "theta"
  Demux1/1 -> Terminator4/1  "phi"
  Spacecraft Dynamics/3 -> [rpy], Demux1/1, Attitude/1  "Vecef"

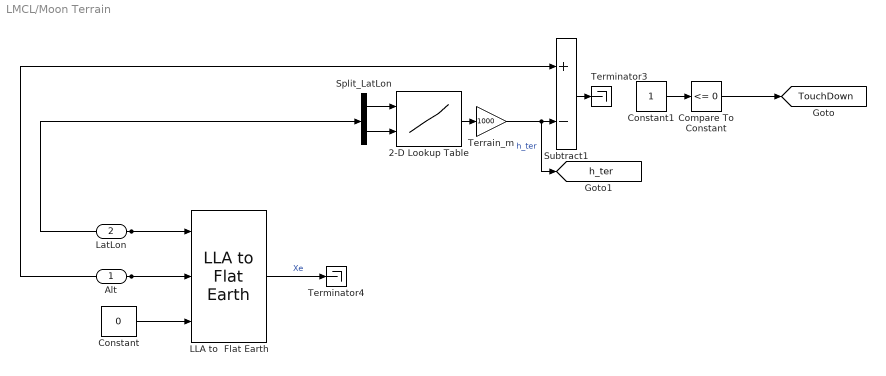
== system LMCL/Moon Terrain ==
  Alt : Inport
  LatLon : Inport  Port=2
  2-D Lookup Table : Lookup_n-D  BreakpointsForDimension1=lat_grid  BreakpointsForDimension2=lon_grid  Table=moon_dem_table  InternalRulePriority=Speed  RndMeth=Simplest
      settings: InputPortMap=u0,u1
  Compare To Constant : simulink/Logic and Bit Operations/Compare To Constant  relop=<=  const=0  OutDataTypeStr=boolean
  Constant : Constant  Value=0
  Constant1 : Constant
  LLA to  Flat Earth : aerolibtransform2/LLA to Flat Earth  units=Metric (MKS)  ptype=Custom  F=0.0012  R=1737.4e3  refPosPort=off  LL0=[-1.13 -141.8]  psi=0
  Split_LatLon : Demux  Outputs=2
  Subtract1 : Sum  Inputs=+-
  Terminator3 : Terminator
  Terminator4 : Terminator
  Terrain_m : Gain  Gain=1000
  tag scope: TouchDown=global, h_ter=global
  wires:
  Alt/1 -> LLA to  Flat Earth/2, Subtract1/1
  LLA to  Flat Earth/1 -> Terminator4/1  "Xe"
  Subtract1/1 -> Terminator3/1
  LatLon/1 -> LLA to  Flat Earth/1, Split_LatLon/1
  Split_LatLon/2 -> 2-D Lookup Table/2
  Constant/1 -> LLA to  Flat Earth/3
  Terrain_m/1 -> [h_ter], Subtract1/2  "h_ter"
  Constant1/1 -> Compare To Constant/1
  Compare To Constant/1 -> [TouchDown]
  Split_LatLon/1 -> 2-D Lookup Table/1
  2-D Lookup Table/1 -> Terrain_m/1

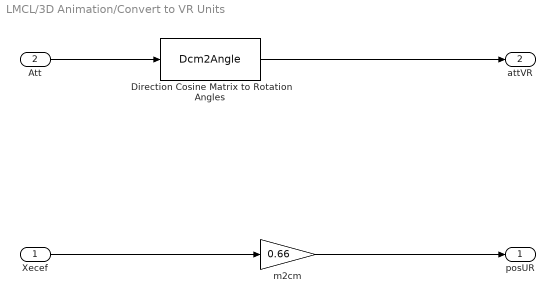
== system LMCL/3D Animation/Convert to VR Units ==
  Xecef : Inport
  Att : Inport  Port=2
  Direction Cosine Matrix to Rotation Angles : Dcm2Angle  rotationOrder=XYZ
      settings: AttributesFormatString=Rotation Order: %<rotationOrder>
  m2cm : Gain  Gain=0.66
  posUR : Outport  VectorParamsAs1DForOutWhenUnconnected=off
  attVR : Outport  Port=2  VectorParamsAs1DForOutWhenUnconnected=off
  wires:
  m2cm/1 -> posUR/1
  Att/1 -> Direction Cosine Matrix to Rotation Angles/1
  Direction Cosine Matrix to Rotation Angles/1 -> attVR/1
  Xecef/1 -> m2cm/1

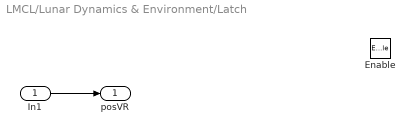
== system LMCL/Lunar Dynamics & Environment/Latch ==
  In1 : Inport
  Enable : EnablePort
  posVR : Outport
  wires:
  In1/1 -> posVR/1

== stateflow chart LMCL/LandingStateMachine ==
  settings: updateMethod=DISCRETE  sampleTime=0.01
  state Orbiting
    entry:
    phase = 1;
    during:
    Fx = 0;
    Fy = 0;
    Fz = 0;
    [ Mx,My,Mz] =AttitudeController(0,0,0,Attitude);
  state BreakOrbit
    en:
    phase = 2;
    during:
    Fx = 0;
    Fy = 0;
    Fz = 1e7;%Breaking Engine Force
    [ Mx,My,Mz] =AttitudeController(0,0,0,Attitude);
  state [Mx,My,Mz] = AttitudeController(PhiCmd,ThtCmd,PsiCmd,Attitude) [function]
  state Hover
    entry:
    phase = 3;
    during:
    [Fx,Fy,Fz] = SpeedController(0,0,0,Velocity);
    [ Mx,My,Mz] =AttitudeController(0,0,0,Attitude);
  state [Fx,Fy,Fz] = SpeedController(VxCmd,VyCmd,VzCmd,Vff) [function]
  state Descent
    entry:
    phase = 4;
    during:
    Fx = 0;
    Fy = 0;
    Fz = AltitudeController(3e3,Altitiude,Velocity)
    [ Mx,My,Mz] =AttitudeController(0,0,0,Attitude);
  state Fz = AltitudeController(AltCmd,Altitude,Vff) [function]
  state ModifyAttitude
    entry:
    phase = 5;
    during:
    Fx = 0;
    Fy = 0;
    Fz = 0;
    [ Mx,My,Mz] =AttitudeController(85,0,0,Attitude);
  state Touchdown
    entry:
    phase = 6;
    during:
    Fx = 0;
    Fy = 0;
    Fz = 0;
    Mx = 0;
    My = 0;
    Mz = 0;
  (default) -> Orbiting
  Orbiting -> BreakOrbit : [after(1,sec)]
  BreakOrbit -> Hover : [after(3.5,sec)]
  Hover -> Descent : [after(70,sec)]
  Descent -> ModifyAttitude : [Altitiude<=4e3 ]
  ModifyAttitude -> Touchdown : [after(2,sec)]
  data: PhiCmd function_input double size=1; ThtCmd function_input double size=1; PsiCmd function_input double size=1; Attitude function_input double size=[3 1]; Mx function_output double size=1; My function_output double size=1; Mz function_output double; VxCmd function_input double size=1; VyCmd function_input double size=1; VzCmd function_input double size=1; Vff function_input double size=[3 1]; Fx function_output double size=1; Fy function_output double size=1; Fz function_output double size=1; AltCmd function_input double size=1; Altitude function_input double size=1; Vff function_input double size=[3 1]; Fz function_output double size=1; Attitude input; Altitiude input; Velocity input; Fx output; Fy output; Fz output; Mx output; My output; Mz output; phase output
